simulink model "AXU5EV_Motor_Control_System"  (R2026b)
settings: Solver=FixedStepDiscrete  StopTime=.0012  FixedStep=2e-8
libraries: AXU5EV_PL_Algorithm_Library x1, AXU5EV_Encoder_Components x1
settings Model: DataTypeOverride=Off  Creator=lww  LastModifiedBy=lww

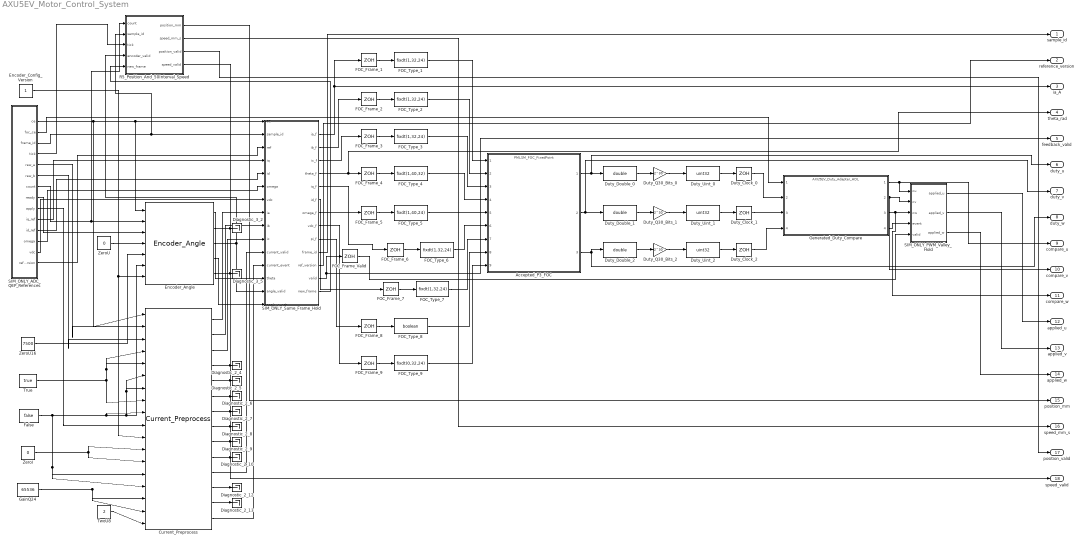
== system AXU5EV_Motor_Control_System ==
  Accepted_P3_FOC : ModelReference  ModelNameDialog=PMLSM_FOC_FixedPoint  SimulationMode=Normal  ModelReferenceVersion=1.16
  Current_Preprocess : AXU5EV_PL_Algorithm_Library/Current_Preprocess  SystemSampleTime=-1  VariantActivationTime=update diagram  EmptyChoice=off  PassThrough=off  PassThroughVariantControl=(default)  EmptyChoiceVariantControl=(default)  AllowFlexibleInterface=on  Latency=0  AutoFrameSizeCalculation=off
  Diagnostic_2_{4..10,12..13} (9 alike) : Terminator
  Diagnostic_3_2 : Terminator
  Diagnostic_3_5 : Terminator
  Duty_Clock_0 : ZeroOrderHold  SampleTime=2e-8
  Duty_Clock_1 : ZeroOrderHold  SampleTime=2e-8
  Duty_Clock_2 : ZeroOrderHold  SampleTime=2e-8
  Duty_Double_0 : DataTypeConversion  OutDataTypeStr=double  SaturateOnIntegerOverflow=off  RndMeth=Floor
  Duty_Double_1 : DataTypeConversion  OutDataTypeStr=double  SaturateOnIntegerOverflow=off  RndMeth=Floor
  Duty_Double_2 : DataTypeConversion  OutDataTypeStr=double  SaturateOnIntegerOverflow=off  RndMeth=Floor
  Duty_Q30_Bits_0 : Gain  Gain=2^30
  Duty_Q30_Bits_1 : Gain  Gain=2^30
  Duty_Q30_Bits_2 : Gain  Gain=2^30
  Duty_Uint_0 : DataTypeConversion  OutDataTypeStr=uint32  RndMeth=Convergent
  Duty_Uint_1 : DataTypeConversion  OutDataTypeStr=uint32  RndMeth=Convergent
  Duty_Uint_2 : DataTypeConversion  OutDataTypeStr=uint32  RndMeth=Convergent
  Encoder_Angle : AXU5EV_Encoder_Components/Encoder_Angle  SystemSampleTime=-1  VariantActivationTime=update diagram  EmptyChoice=off  PassThrough=off  PassThroughVariantControl=(default)  EmptyChoiceVariantControl=(default)  AllowFlexibleInterface=on  Latency=0  AutoFrameSizeCalculation=off
  Encoder_Config_Version : Constant  OutDataTypeStr=uint32  SampleTime=2e-8
  FOC_Frame_{1..9} (9 alike) : ZeroOrderHold  SampleTime=1e-4
  FOC_Frame_Valid : ZeroOrderHold  SampleTime=1e-4
  FOC_Type_{1..3,6..7} (5 alike) : DataTypeConversion  OutDataTypeStr=fixdt(1,32,24)  RndMeth=Convergent
  FOC_Type_4 : DataTypeConversion  OutDataTypeStr=fixdt(1,40,32)  RndMeth=Convergent
  FOC_Type_5 : DataTypeConversion  OutDataTypeStr=fixdt(1,40,24)  RndMeth=Convergent
  FOC_Type_8 : DataTypeConversion  OutDataTypeStr=boolean  RndMeth=Convergent
  FOC_Type_9 : DataTypeConversion  OutDataTypeStr=fixdt(0,32,24)  RndMeth=Convergent
  False : Constant  Value=false  OutDataTypeStr=boolean  SampleTime=2e-8
  GainQ24 : Constant  Value=65536  OutDataTypeStr=int32  SampleTime=2e-8
  Generated_Duty_Compare : ModelReference  ModelNameDialog=AXU5EV_Duty_Adapter_HDL  SimulationMode=Normal  ModelReferenceVersion=1.2
  R5_Position_And_50Interval_Speed : MATLAB Function  TreatAsAtomicUnit=on
  SIM_ONLY_ADC_QEP_References : MATLAB Function  TreatAsAtomicUnit=on
  SIM_ONLY_PWM_Valley_Hold : MATLAB Function  TreatAsAtomicUnit=on
  SIM_ONLY_Same_Frame_Hold : MATLAB Function  TreatAsAtomicUnit=on
  True : Constant  Value=true  OutDataTypeStr=boolean  SampleTime=2e-8
  TwoU8 : Constant  Value=2  OutDataTypeStr=uint8  SampleTime=2e-8
  ZeroI : Constant  Value=0  OutDataTypeStr=int32  SampleTime=2e-8
  ZeroU : Constant  Value=0  OutDataTypeStr=uint32  SampleTime=2e-8
  ZeroU16 : Constant  Value=7500  OutDataTypeStr=uint16  SampleTime=2e-8
  sample_id : Outport
  reference_version : Outport  Port=2
  ia_A : Outport  Port=3
  theta_rad : Outport  Port=4
  feedback_valid : Outport  Port=5
  duty_u : Outport  Port=6
  duty_v : Outport  Port=7
  duty_w : Outport  Port=8
  compare_u : Outport  Port=9
  compare_v : Outport  Port=10
  compare_w : Outport  Port=11
  applied_u : Outport  Port=12
  applied_v : Outport  Port=13
  applied_w : Outport  Port=14
  position_mm : Outport  Port=15
  speed_mm_s : Outport  Port=16
  position_valid : Outport  Port=17
  speed_valid : Outport  Port=18
  wires:
  FOC_Frame_9/1 -> FOC_Type_9/1
  SIM_ONLY_Same_Frame_Hold/8(vdc_f) -> FOC_Frame_9/1
  FOC_Frame_8/1 -> FOC_Type_8/1
  SIM_ONLY_Same_Frame_Hold/9(pi_f) -> FOC_Frame_8/1
  FOC_Frame_5/1 -> FOC_Type_5/1
  SIM_ONLY_Same_Frame_Hold/7(omega_f) -> FOC_Frame_5/1
  FOC_Frame_4/1 -> FOC_Type_4/1
  SIM_ONLY_Same_Frame_Hold/4(theta_f) -> theta_rad/1, FOC_Frame_4/1
  FOC_Frame_3/1 -> FOC_Type_3/1
  SIM_ONLY_Same_Frame_Hold/3(ic_f) -> FOC_Frame_3/1
  FOC_Frame_2/1 -> FOC_Type_2/1
  SIM_ONLY_Same_Frame_Hold/2(ib_f) -> FOC_Frame_2/1
  FOC_Frame_1/1 -> FOC_Type_1/1
  SIM_ONLY_Same_Frame_Hold/1(ia_f) -> FOC_Frame_1/1, ia_A/1
  Encoder_Angle/4 -> SIM_ONLY_Same_Frame_Hold/15(angle_event)
  Encoder_Angle/3 -> SIM_ONLY_Same_Frame_Hold/14(angle_valid), R5_Position_And_50Interval_Speed/4(encoder_valid)
  Encoder_Angle/1 -> SIM_ONLY_Same_Frame_Hold/13(theta)
  Current_Preprocess/14 -> SIM_ONLY_Same_Frame_Hold/12(current_event)
  Current_Preprocess/11 -> SIM_ONLY_Same_Frame_Hold/11(current_valid)
  Current_Preprocess/3 -> SIM_ONLY_Same_Frame_Hold/10(ic)
  Current_Preprocess/2 -> SIM_ONLY_Same_Frame_Hold/9(ib)
  Current_Preprocess/1 -> SIM_ONLY_Same_Frame_Hold/8(ia)
  SIM_ONLY_ADC_QEP_References/13(vdc) -> SIM_ONLY_Same_Frame_Hold/7(vdc)
  SIM_ONLY_ADC_QEP_References/12(omega) -> SIM_ONLY_Same_Frame_Hold/6(omega)
  SIM_ONLY_ADC_QEP_References/11(id_ref) -> SIM_ONLY_Same_Frame_Hold/5(id)
  SIM_ONLY_ADC_QEP_References/10(iq_ref) -> SIM_ONLY_Same_Frame_Hold/4(iq)
  SIM_ONLY_ADC_QEP_References/3(frame_id) -> R5_Position_And_50Interval_Speed/2(sample_id), SIM_ONLY_Same_Frame_Hold/2(sample_id)
  ZeroU16/1 -> Encoder_Angle/5
  ZeroU/1 -> Encoder_Angle/4
  SIM_ONLY_ADC_QEP_References/8(ready) -> Encoder_Angle/3
  SIM_ONLY_ADC_QEP_References/7(count) -> R5_Position_And_50Interval_Speed/1(count), Encoder_Angle/2
  TwoU8/1 -> Current_Preprocess/18
  GainQ24/1 -> Current_Preprocess/16, Current_Preprocess/17
  ZeroI/1 -> Current_Preprocess/12, Current_Preprocess/13
  SIM_ONLY_ADC_QEP_References/14(ref_version) -> SIM_ONLY_Same_Frame_Hold/3(ref)
  SIM_ONLY_ADC_QEP_References/9(apply) -> Current_Preprocess/10
  False/1 -> Current_Preprocess/14, Current_Preprocess/15, Current_Preprocess/6, Current_Preprocess/7, Encoder_Angle/6, Current_Preprocess/9
  True/1 -> Current_Preprocess/4, Current_Preprocess/5, Current_Preprocess/8
  SIM_ONLY_ADC_QEP_References/6(raw_b) -> Current_Preprocess/3
  SIM_ONLY_ADC_QEP_References/5(raw_a) -> Current_Preprocess/2
  SIM_ONLY_ADC_QEP_References/1(ce) -> SIM_ONLY_Same_Frame_Hold/1(ce), Encoder_Angle/1, Current_Preprocess/1
  Encoder_Config_Version/1 -> Encoder_Angle/7, Current_Preprocess/11
  SIM_ONLY_Same_Frame_Hold/10(frame_id) -> sample_id/1
  SIM_ONLY_Same_Frame_Hold/11(ref_version) -> reference_version/1
  Current_Preprocess/4 -> Diagnostic_2_4/1
  Current_Preprocess/5 -> Diagnostic_2_5/1
  Current_Preprocess/6 -> Diagnostic_2_6/1
  Current_Preprocess/7 -> Diagnostic_2_7/1
  Current_Preprocess/8 -> Diagnostic_2_8/1
  Current_Preprocess/9 -> Diagnostic_2_9/1
  Current_Preprocess/10 -> Diagnostic_2_10/1
  Current_Preprocess/12 -> Diagnostic_2_12/1
  Current_Preprocess/13 -> Diagnostic_2_13/1
  Encoder_Angle/2 -> Diagnostic_3_2/1
  Encoder_Angle/5 -> Diagnostic_3_5/1
  SIM_ONLY_ADC_QEP_References/4(tick) -> R5_Position_And_50Interval_Speed/3(tick)
  SIM_ONLY_Same_Frame_Hold/13(new_frame) -> R5_Position_And_50Interval_Speed/5(new_frame)
  R5_Position_And_50Interval_Speed/1(position_mm) -> position_mm/1
  R5_Position_And_50Interval_Speed/2(speed_mm_s) -> speed_mm_s/1
  R5_Position_And_50Interval_Speed/3(position_valid) -> position_valid/1
  R5_Position_And_50Interval_Speed/4(speed_valid) -> speed_valid/1
  FOC_Frame_Valid/1 -> SIM_ONLY_PWM_Valley_Hold/5(valid)
  SIM_ONLY_PWM_Valley_Hold/3(applied_w) -> applied_w/1
  SIM_ONLY_PWM_Valley_Hold/2(applied_v) -> applied_v/1
  SIM_ONLY_PWM_Valley_Hold/1(applied_u) -> applied_u/1
  FOC_Type_1/1 -> Accepted_P3_FOC/1
  FOC_Type_2/1 -> Accepted_P3_FOC/2
  FOC_Type_3/1 -> Accepted_P3_FOC/3
  FOC_Type_4/1 -> Accepted_P3_FOC/4
  FOC_Type_5/1 -> Accepted_P3_FOC/5
  SIM_ONLY_Same_Frame_Hold/5(iq_f) -> FOC_Frame_6/1
  FOC_Frame_6/1 -> FOC_Type_6/1
  FOC_Type_6/1 -> Accepted_P3_FOC/6
  SIM_ONLY_Same_Frame_Hold/6(id_f) -> FOC_Frame_7/1
  FOC_Frame_7/1 -> FOC_Type_7/1
  FOC_Type_7/1 -> Accepted_P3_FOC/7
  FOC_Type_8/1 -> Accepted_P3_FOC/8
  FOC_Type_9/1 -> Accepted_P3_FOC/9
  Accepted_P3_FOC/1 -> duty_u/1, Duty_Double_0/1
  Duty_Double_0/1 -> Duty_Q30_Bits_0/1
  Duty_Q30_Bits_0/1 -> Duty_Uint_0/1
  Duty_Uint_0/1 -> Duty_Clock_0/1
  Duty_Clock_0/1 -> Generated_Duty_Compare/2
  Generated_Duty_Compare/1 -> compare_u/1, SIM_ONLY_PWM_Valley_Hold/1(cu)
  Accepted_P3_FOC/2 -> duty_v/1, Duty_Double_1/1
  Duty_Double_1/1 -> Duty_Q30_Bits_1/1
  Duty_Q30_Bits_1/1 -> Duty_Uint_1/1
  Duty_Uint_1/1 -> Duty_Clock_1/1
  Duty_Clock_1/1 -> Generated_Duty_Compare/3
  Generated_Duty_Compare/2 -> SIM_ONLY_PWM_Valley_Hold/2(cv), compare_v/1
  Accepted_P3_FOC/3 -> Duty_Double_2/1, duty_w/1
  Duty_Double_2/1 -> Duty_Q30_Bits_2/1
  Duty_Q30_Bits_2/1 -> Duty_Uint_2/1
  Duty_Uint_2/1 -> Duty_Clock_2/1
  Duty_Clock_2/1 -> Generated_Duty_Compare/4
  Generated_Duty_Compare/3 -> compare_w/1, SIM_ONLY_PWM_Valley_Hold/3(cw)
  SIM_ONLY_ADC_QEP_References/2(foc_ce) -> Generated_Duty_Compare/1
  Generated_Duty_Compare/4 -> SIM_ONLY_PWM_Valley_Hold/4(event)
  SIM_ONLY_Same_Frame_Hold/12(valid) -> FOC_Frame_Valid/1, feedback_valid/1

== matlab function AXU5EV_Motor_Control_System/SIM_ONLY_Same_Frame_Hold ==
  data: ce input; ia_f output; sample_id input; ref input; iq input; id input; omega input; vdc input; ia input; ib input; ic input; current_valid input; current_event input; theta input; angle_valid input; angle_event input; ib_f output; ic_f output; theta_f output; iq_f output; id_f output; omega_f output; vdc_f output; pi_f output; frame_id output; ref_version output; valid output; new_frame output
function [ia_f,ib_f,ic_f,theta_f,iq_f,id_f,omega_f,vdc_f,pi_f,frame_id,ref_version,valid,new_frame]=f(ce,sample_id,ref,iq,id,omega,vdc,ia,ib,ic,current_valid,current_event,theta,angle_valid,angle_event)
[ia_f,ib_f,ic_f,theta_f,iq_f,id_f,omega_f,vdc_f,pi_f,frame_id,ref_version,valid,new_frame]=motor_control_sim_join(ce,sample_id,ref,iq,id,omega,vdc,ia,ib,ic,current_valid,current_event,theta,angle_valid,angle_event);
end

== matlab function AXU5EV_Motor_Control_System/SIM_ONLY_ADC_QEP_References ==
  data: ce output; foc_ce output; frame_id output; tick output; raw_a output; raw_b output; count output; ready output; apply output; iq_ref output; id_ref output; omega output; vdc output; ref_version output
function [ce,foc_ce,frame_id,tick,raw_a,raw_b,count,ready,apply,iq_ref,id_ref,omega,vdc,ref_version]=f()
[ce,foc_ce,frame_id,tick,raw_a,raw_b,count,ready,apply,iq_ref,id_ref,omega,vdc,ref_version]=motor_control_sim_io();
end

== matlab function AXU5EV_Motor_Control_System/SIM_ONLY_PWM_Valley_Hold ==
  data: cu input; applied_u output; cv input; cw input; event input; valid input; applied_v output; applied_w output
function [applied_u,applied_v,applied_w]=f(cu,cv,cw,event,valid)
[applied_u,applied_v,applied_w]=motor_control_sim_pwm(cu,cv,cw,event,valid);
end

== matlab function AXU5EV_Motor_Control_System/R5_Position_And_50Interval_Speed ==
  data: count input; position_mm output; sample_id input; tick input; encoder_valid input; new_frame input; speed_mm_s output; position_valid output; speed_valid output
function [position_mm,speed_mm_s,position_valid,speed_valid]=f(count,sample_id,tick,encoder_valid,new_frame)
[position_mm,speed_mm_s,position_valid,speed_valid]=motor_control_sim_r5(count,sample_id,tick,encoder_valid,new_frame);
end
